simulink library "focLib"  (R2023a)
settings: Solver=VariableStepAuto  StartTime=0.0  StopTime=10.0  RelTol=1e-3
undefined symbols (not defined in the file): availableSpeedModes, ctrl_limits, Down, focp_tune_cur_Ki, focp_tune_cur_Kp, focp_tune_iq_max, focp_tune_iq_min, focp_tune_spd_Ki, focp_tune_spd_Kp, focp_tune_udc_max, GPTRIP1SEL, inverter_DRV8300, PI_params, pmsm_ECI6360, PU_System, target_f2838, Ts, Ts_motor, Ts_simulink, Ts_speed, TZ1, Up
libraries: simulink x31, c2802xlib x12, idelinklib_common x8, mcbcontrolslib x8, c280xlib x7, mcbpositiondecoderlib x7, slpidlib x5, c2837xDlib x2, c2838xlib x1, autolibpmsminterior x1, mcbplantlib x1, autolibpmsmexterior x1
(part 3 of 3)

== system focLib/Torque Controller/FOC/Current_Controllers/PI_Controller_Iq ==
  Iq_in : Inport
  Data Store Read1 : DataStoreRead  Commented=on  DataStoreName=Enable  IndexOptions=Index vector (dialog)  Indices=1  OutputSizes=1
  Discrete PI Controller with anti-windup & reset : slpidlib/PID Controller  Commented=on  Controller=PI  Form=Parallel  TimeDomain=Discrete-time  UseExternalTs=off  SampleTime=-1  IntegratorMethod=Forward Euler  FilterMethod=Forward Euler  ControllerParametersSource=external  P=1  I=1  UseKiTs=on  D=0  N=100  UseFilter=on  TunerSelectOption=Transfer Function Based (PID Tuner App)  InitialConditionSource=external  InitialConditionForIntegrator=0  InitialConditionForFilter=0  DifferentiatorICPrevScaledInput=0  ExternalReset=level  TrackingMode=off  Kt=1  LimitOutput=on  SatLimitsSource=internal  UpperSaturationLimit=1  LowerSaturationLimit=-1  LinearizeAsGain=on  AntiWindupMode=clamping  Kb=1  LimitIntegrator=off  UpperIntegratorSaturationLimit=inf  LowerIntegratorSaturationLimit=-inf  RndMeth=Simplest  POutMin=[]  POutMax=[]  IOutMin=[]  IOutMax=[]  DOutMin=[]  DOutMax=[]  NOutMin=[]  NOutMax=[]  SumOutMin=[]  SumOutMax=[]  SaturationOutDataTypeStr=Inherit: Inherit via back propagation  SaturationOutMin=[]  SaturationOutMax=[]  PParamMin=[]  PParamMax=[]  IParamMin=[]  IParamMax=[]  DParamMin=[]  DParamMax=[]  NParamMin=[]  NParamMax=[]  KbParamMin=[]  KbParamMax=[]  KtParamMin=[]  KtParamMax=[]  KbOutMin=[]  KbOutMax=[]  KtOutMin=[]  KtOutMax=[]  IntegratorOutMin=[]  IntegratorOutMax=[]  FilterOutMin=[]  FilterOutMax=[]  SumI1OutMin=[]  SumI1OutMax=[]  SumI2OutMin=[]  SumI2OutMax=[]  SumI3OutMin=[]  SumI3OutMax=[]  SumI4OutMin=[]  SumI4OutMax=[]  SumDOutMin=[]  SumDOutMax=[]  DifferentiatorOutMin=[]  DifferentiatorOutMax=[]  FilterDiffOutCoefMin=[]  FilterDiffOutCoefMax=[]  ReciprocalOutMin=[]  ReciprocalOutMax=[]  SumDenOutMin=[]  SumDenOutMax=[]  SumNumOutMin=[]  SumNumOutMax=[]  DivideOutMin=[]  DivideOutMax=[]  UdiffTsProdOutMin=[]  UdiffTsProdOutMax=[]  NTsProdOutMin=[]  NTsProdOutMax=[]  UintegralTsProdOutMin=[]  UintegralTsProdOutMax=[]  UngainTsProdOutMin=[]  UngainTsProdOutMax=[]  ClampingZeroOutDataTypeStr=Inherit: Inherit via back propagation  ClampingZeroOutMin=[]  ClampingZeroOutMax=[]  FilterDenConstantOutDataTypeStr=Inherit: Inherit via back propagation  FilterDenConstantOutMin=[]  FilterDenConstantOutMax=[]  PCopyOutDataTypeStr=Inherit: Inherit via back propagation  PCopyOutMin=[]  PCopyOutMax=[]  NCopyOutDataTypeStr=Inherit: Inherit via back propagation  NCopyOutMin=[]  NCopyOutMax=[]  IntegratorContinuousStateAttributes=''  IntegratorStateMustResolveToSignalObject=off  IntegratorRTWStateStorageClass=Auto  FilterContinuousStateAttributes=''  FilterStateMustResolveToSignalObject=off  FilterRTWStateStorageClass=Auto  ParallelPVariant=ExternalParameters  IdealPVariant=Disabled  IVariant=ExternalParameters  DVariant=Disabled  IntegratorVariant=Discrete  SatVariant=Enabled  AWVariant=DiscClampingParallel  PCopyVariant=Disabled  TRVariant=Disabled  FdbkBlocksVariant=Forward  IdealPFdbkVariant=Disabled  SatFdbkVariant=Disabled  DerivativeFilterVariant=Disabled  NVariant=Disabled  NCopyVariant=Disabled_SignalSpec  FilterICVariant=Disabled  IntegratorICVariant=ExternalICs  ExternalResetVariant=ExternalReset  TRSumVariant=Passthrough  SumFdbkVariant=Disabled  SumVariant=Sum_PI  TsampFilterVariant=InternalTs  TsampNgainVariant=Passthrough  TsampIntegralVariant=Disabled_SignalSpec  ExternalSaturationOutDataTypeStr=Inherit: Same as second input
      settings: LibrarySourceBlock=mcbcontrolslib/PI Controller
  Ki : Constant  Commented=on  Value=PI_params.Ki_i*Ts  OutDataTypeStr=single  SampleTime=-1
  Kp : Constant  Commented=on  Value=PI_params.Kp_i  OutDataTypeStr=single  SampleTime=-1
  Kp1 : Constant  Commented=on  Value=0  OutDataTypeStr=single  SampleTime=-1
  Logical Operator : Logic  Commented=on  Operator=NOT  IconShape=distinctive  AllPortsSameDT=off  OutDataTypeStr=boolean
  PID Controller : slpidlib/PID Controller  Controller=PI  Form=Parallel  TimeDomain=Discrete-time  UseExternalTs=off  SampleTime=-1  IntegratorMethod=Forward Euler  FilterMethod=Forward Euler  ControllerParametersSource=internal  P=focp_tune_cur_Kp  I=focp_tune_cur_Ki  UseKiTs=off  D=0  N=100  UseFilter=on  TunerSelectOption=Transfer Function Based (PID Tuner App)  InitialConditionSource=internal  InitialConditionForIntegrator=0  InitialConditionForFilter=0  DifferentiatorICPrevScaledInput=0  ExternalReset=level  TrackingMode=off  Kt=1  LimitOutput=on  SatLimitsSource=internal  UpperSaturationLimit=1  LowerSaturationLimit=-1  LinearizeAsGain=off  AntiWindupMode=clamping  Kb=1  LimitIntegrator=off  UpperIntegratorSaturationLimit=inf  LowerIntegratorSaturationLimit=-inf  POutMin=[]  POutMax=[]  IOutMin=[]  IOutMax=[]  DOutMin=[]  DOutMax=[]  NOutMin=[]  NOutMax=[]  SumOutMin=[]  SumOutMax=[]  SaturationOutMin=[]  SaturationOutMax=[]  PParamDataTypeStr=fixdt(1,32,24)  PParamMin=[]  PParamMax=[]  IParamDataTypeStr=fixdt(1,32,16)  IParamMin=[]  IParamMax=[]  DParamMin=[]  DParamMax=[]  NParamMin=[]  NParamMax=[]  KbParamMin=[]  KbParamMax=[]  KtParamMin=[]  KtParamMax=[]  KbOutMin=[]  KbOutMax=[]  KtOutMin=[]  KtOutMax=[]  IntegratorOutMin=[]  IntegratorOutMax=[]  FilterOutMin=[]  FilterOutMax=[]  SumI1OutMin=[]  SumI1OutMax=[]  SumI2OutMin=[]  SumI2OutMax=[]  SumI3OutMin=[]  SumI3OutMax=[]  SumI4OutMin=[]  SumI4OutMax=[]  SumDOutMin=[]  SumDOutMax=[]  DifferentiatorOutMin=[]  DifferentiatorOutMax=[]  FilterDiffOutCoefMin=[]  FilterDiffOutCoefMax=[]  ReciprocalOutMin=[]  ReciprocalOutMax=[]  SumDenOutMin=[]  SumDenOutMax=[]  SumNumOutMin=[]  SumNumOutMax=[]  DivideOutMin=[]  DivideOutMax=[]  UdiffTsProdOutMin=[]  UdiffTsProdOutMax=[]  NTsProdOutMin=[]  NTsProdOutMax=[]  UintegralTsProdOutMin=[]  UintegralTsProdOutMax=[]  UngainTsProdOutMin=[]  UngainTsProdOutMax=[]  ClampingZeroOutDataTypeStr=Inherit: Inherit via back propagation  ClampingZeroOutMin=[]  ClampingZeroOutMax=[]  FilterDenConstantOutDataTypeStr=Inherit: Inherit via back propagation  FilterDenConstantOutMin=[]  FilterDenConstantOutMax=[]  PCopyOutDataTypeStr=Inherit: Inherit via back propagation  PCopyOutMin=[]  PCopyOutMax=[]  NCopyOutDataTypeStr=Inherit: Inherit via back propagation  NCopyOutMin=[]  NCopyOutMax=[]  IntegratorContinuousStateAttributes=''  IntegratorStateMustResolveToSignalObject=off  IntegratorRTWStateStorageClass=Auto  FilterContinuousStateAttributes=''  FilterStateMustResolveToSignalObject=off  FilterRTWStateStorageClass=Auto  ParallelPVariant=InternalParameters  IdealPVariant=Disabled  IVariant=InternalParameters  DVariant=Disabled  IntegratorVariant=Discrete  SatVariant=Enabled  AWVariant=DiscClampingParallel  PCopyVariant=Disabled  TRVariant=Disabled  FdbkBlocksVariant=Forward  IdealPFdbkVariant=Disabled  SatFdbkVariant=Disabled  DerivativeFilterVariant=Disabled  NVariant=Disabled  NCopyVariant=Disabled_SignalSpec  FilterICVariant=Disabled  IntegratorICVariant=InternalICs  ExternalResetVariant=ExternalReset  TRSumVariant=Passthrough  SumFdbkVariant=Disabled  SumVariant=Sum_PI  TsampFilterVariant=InternalTs  TsampNgainVariant=Passthrough  TsampIntegralVariant=Disabled_SignalSpec  ExternalSaturationOutDataTypeStr=Inherit: Same as second input
  Reset_I_Cur_And : Logic  AllPortsSameDT=off  OutDataTypeStr=boolean
  Reset_I_Cur_Enable : Constant  Value=ctrl_limits.reset_I_cur_freemode  OutDataTypeStr=boolean
  V_ref : Outport  VectorParamsAs1DForOutWhenUnconnected=off
  wires:
  Iq_in/1 -> PID Controller/1
  PID Controller/1 -> V_ref/1
  Kp1/1 -> Discrete PI Controller with anti-windup & reset/5
  Logical Operator/1 -> Discrete PI Controller with anti-windup & reset/4
  Ki/1 -> Discrete PI Controller with anti-windup & reset/3
  Kp/1 -> Discrete PI Controller with anti-windup & reset/2
  Data Store Read1/1 -> Logical Operator/1
  [FreemodeSig_I] -> Reset_I_Cur_And/1
  Reset_I_Cur_Enable/1 -> Reset_I_Cur_And/2
  Reset_I_Cur_And/1 -> PID Controller/2

== system focLib/Torque Controller/Input Scaling/CodeGeneration/Calculate Position from Hall ==
  Atomic Hall Reading : Subsystem
  Data Store Write : DataStoreWrite  DataStoreName=HallStateChangeFlag  IndexOptions=Index vector (dialog)  Indices=1  OutputSizes=1
  Glitch Filter : simulink/Logic and Bit Operations/Compare To Constant  relop=>=  const=target_f2838.CPU_frequency * 600 / (pmsm_ECI6360.N_base * 10 * 2 * pmsm_ECI6360.p)  OutDataTypeStr=boolean
  Hall Speed and Position : mcbpositiondecoderlib/Hall Speed and Position  blkExecutionType=Speed and position  CounterSize=32 bits  ClkFreq=target_f2838.CPU_frequency  BlkSampleTime=Ts  PolePairs=pmsm_ECI6360.p  MinSpeed=20  HallInterruptConfig=Every 180 Degrees  SpeedUnit=Per unit  PerUnitSpeed=PU_System.N_base  SpeedDataType=fixdt(1,32,17)  hallSequence=ABC  Sequence=[5,4,6,2,3,1]  EnableSecondOrder=1st Order  PositionUnit=Per unit  PositionDataType=fixdt(1,32,17)
      settings: LibrarySourceBlock=mcblib/Sensor Decoders/Hall Speed and Position
  Mechanical to Electrical Position : mcbpositiondecoderlib/Mechanical to Electrical Position  NrPP=1  selectedRange=Per unit  MechOfstInputType=Specify via dialog  mechOffsetIn=0.38  maxAngleIn=1  InputDataType=fixdt(1,32,17)  VariantSelect=floating-point
      settings: LibrarySourceBlock=mcblib/Sensor Decoders/Mechanical to Electrical Position
  Subsystem : Subsystem
  Pos_PU : Outport
  Speed_PU : Outport  Port=2
  wires:
  Hall Speed and Position/2 -> Speed_PU/1
  Subsystem/1(Output) -> Hall Speed and Position/3
  Atomic Hall Reading/3(SpeedCount) -> Glitch Filter/1, Subsystem/1(Input)
  Glitch Filter/1 -> Subsystem/Enable
  Mechanical to Electrical Position/1 -> Pos_PU/1
  Hall Speed and Position/1 -> Mechanical to Electrical Position/1
  Atomic Hall Reading/1(HallState) -> Hall Speed and Position/1
  Atomic Hall Reading/4(Direction) -> Hall Speed and Position/4
  Atomic Hall Reading/2(Count) -> Hall Speed and Position/2
  Atomic Hall Reading/5(SpeedValidity) -> Hall Speed and Position/5
  Hall Speed and Position/3 -> Data Store Write/1
  Atomic Hall Reading/6(HallChange) -> Hall Speed and Position/6

== system focLib/Torque Controller/Input Scaling/CodeGeneration/Convert ADC value to PU ==
  note: Shift Gain mit 2hoch9 und fixdt(1,32,20) einmal versuchen
  Iab_ADC : Inport
  Add : Sum  Inputs=+-
  Data Store Read : DataStoreRead  DataStoreName=IaOffset  IndexOptions=Index vector (dialog)  Indices=1  OutputSizes=1
  Data Store Read1 : DataStoreRead  DataStoreName=IbOffset  IndexOptions=Index vector (dialog)  Indices=1  OutputSizes=1
  Data Type Conversion : DataTypeConversion  OutDataTypeStr=int32  ConvertRealWorld=Stored Integer (SI)  SaturateOnIntegerOverflow=off  RndMeth=Floor
  Data Type Conversion1 : DataTypeConversion  OutDataTypeStr=fixdt(1,32,17)  ConvertRealWorld=Stored Integer (SI)  SaturateOnIntegerOverflow=off  RndMeth=Floor
  Display{,1..3} (4 alike) : Display
  Mux : Mux  Inputs=2
  Shift Arithmetic : ArithShift  BitShiftNumber=-6
  Iab_PU : Outport
  wires:
  Data Store Read1/1 -> Mux/2
  Data Store Read/1 -> Mux/1
  Data Type Conversion1/1 -> Display/1, Iab_PU/1
  Shift Arithmetic/1 -> Data Type Conversion1/1, Display1/1
  Add/1 -> Shift Arithmetic/1, Display2/1
  Mux/1 -> Add/2
  Data Type Conversion/1 -> Add/1, Display3/1
  Iab_ADC/1 -> Data Type Conversion/1

== system focLib/Torque Controller/Input Scaling/Simulation/Convert Iab to PU ==
  Iab_ADC_Sim : Inport
  Add : Sum  Inputs=+-
  Constant : Constant  Value=[inverter_DRV8300.CtSensAOffset inverter_DRV8300.CtSensBOffset]  SampleTime=-1
  Current Sense Gain : Gain  Commented=on  Gain=PU_System.I_base/1.65  RndMeth=Simplest  OutDataTypeStr=Inherit: Same as input
  Data Type Conversion : DataTypeConversion  OutDataTypeStr=int32  ConvertRealWorld=Stored Integer (SI)  SaturateOnIntegerOverflow=off  RndMeth=Floor
  Data Type Conversion1 : DataTypeConversion  OutDataTypeStr=fixdt(1,32,17)  ConvertRealWorld=Stored Integer (SI)  RndMeth=Simplest  SaturateOnIntegerOverflow=off
  Get_ADC_Volt : Gain  Commented=on  Gain=1.65/(4096/2)  OutDataTypeStr=double  RndMeth=Simplest
  PU_Conversion : Gain  Commented=on  Gain=1/PU_System.I_base  RndMeth=Simplest  OutDataTypeStr=Inherit: Same as input
  Shift Arithmetic : ArithShift  BitShiftNumber=-6
  Iab_PU : Outport
  wires:
  Get_ADC_Volt/1 -> Current Sense Gain/1
  Current Sense Gain/1 -> PU_Conversion/1
  Add/1 -> Shift Arithmetic/1
  Shift Arithmetic/1 -> Data Type Conversion1/1
  Data Type Conversion1/1 -> Iab_PU/1
  Constant/1 -> Add/2
  Data Type Conversion/1 -> Add/1
  Iab_ADC_Sim/1 -> Data Type Conversion/1

== system focLib/Torque Controller/Input Scaling/Simulation/Convert Pos to PU ==
  Pos_Sim : Inport
  IIR Filter : mcbcontrolslib/IIR Filter  VariantControl=Low Pass Filter  VariantSelect=Low-pass  Filter_constant=0.2  advancedSettings=off  Ts=50e-6  cutOff_freq=795.7747
      settings: LibrarySourceBlock=mcbhdllib/Signal Management/IIR Filter
  Mechanical to Electrical Position : mcbpositiondecoderlib/Mechanical to Electrical Position  NrPP=pmsm_ECI6360.p  selectedRange=Per unit  MechOfstInputType=Specify via dialog  mechOffsetIn=0.38  maxAngleIn=1  InputDataType=fixdt(1,32,17)  VariantSelect=floating-point
      settings: LibrarySourceBlock=mcblib/Sensor Decoders/Mechanical to Electrical Position
  Speed Measurement : mcbpositiondecoderlib/Speed Measurement  PositionUnit=Per unit  PositionScalingDatatype=uint32  SpeedCalculationMode=Time interval for speed calculation  SampleTimeAsync=Ts  MaximumApplicationSpeed=1000  SpeedResolution=5e-6  DelayLength=10  MaximumMeasurableSpeed=59999  MeasurableSpeedResolution=2.794e-05  SpeedUnit=Per unit based on dialog  PerUnitSpeed=PU_System.N_base  SpeedDataType=fixdt(1,32,17)
      settings: LibrarySourceBlock=mcblib/Sensor Decoders/Speed Measurement
  Theta : Outport
  Speed_PU : Outport  Port=2
  wires:
  IIR Filter/1 -> Speed_PU/1
  Mechanical to Electrical Position/1 -> Theta/1
  Speed Measurement/1 -> IIR Filter/1
  Pos_Sim/1 -> Speed Measurement/1, Mechanical to Electrical Position/1

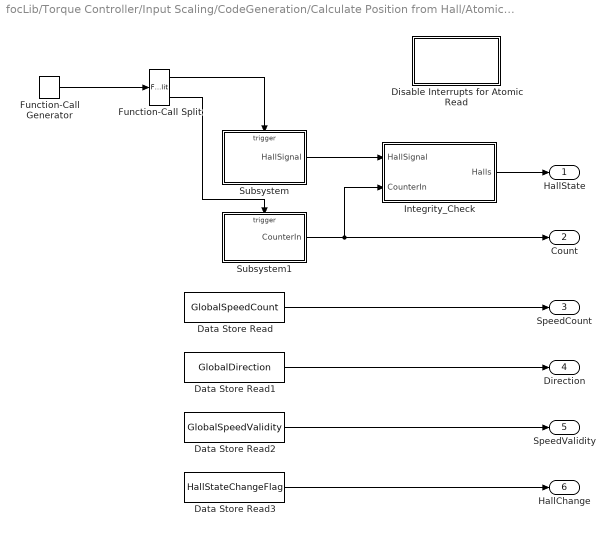
== system focLib/Torque Controller/Input Scaling/CodeGeneration/Calculate Position from Hall/Atomic Hall Reading ==
  Data Store Read : DataStoreRead  DataStoreName=GlobalSpeedCount  IndexOptions=Index vector (dialog)  Indices=1  OutputSizes=1
  Data Store Read1 : DataStoreRead  DataStoreName=GlobalDirection  IndexOptions=Index vector (dialog)  Indices=1  OutputSizes=1
  Data Store Read2 : DataStoreRead  DataStoreName=GlobalSpeedValidity  IndexOptions=Index vector (dialog)  Indices=1  OutputSizes=1
  Data Store Read3 : DataStoreRead  DataStoreName=HallStateChangeFlag  IndexOptions=Index vector (dialog)  Indices=1  OutputSizes=1
  Disable Interrupts for Atomic Read : Subsystem  mask(System Outputs){ShowInLibBrowser=0}
      mask prompts: ShowInLibBrowser "Simulink:masks:CustCodeMaskParam1_MP"
      settings: CopyFcn=cccopyfcn(gcb)  OpenFcn=ccopenfcn('System Outputs Function')
      mask Help: eval('feval(''rtwprivate'',''rtwhelpview'',''rtw_sys_outputs_block'')');
      mask Display: disp('System\nOutputs');
  Function-Call Generator : simulink/Ports & Subsystems/Function-Call Generator  sample_time=-1  numberOfIterations=1  DisallowWideOutput=off
  Function-Call Split : FunctionCallSplit  IconShape=distinctive  NumOutputPorts=2  OutputPortLayout=default
  Integrity_Check : Subsystem
  Subsystem : Subsystem
  Subsystem1 : Subsystem
  HallState : Outport
  Count : Outport  Port=2
  SpeedCount : Outport  Port=3
  Direction : Outport  Port=4
  SpeedValidity : Outport  Port=5
  HallChange : Outport  Port=6
  wires:
  Subsystem1/1(CounterIn) -> Integrity_Check/2(CounterIn), Count/1
  Function-Call Split/1 -> Subsystem/Trigger
  Function-Call Split/2 -> Subsystem1/Trigger
  Integrity_Check/1(Halls) -> HallState/1
  Subsystem/1(HallSignal) -> Integrity_Check/1(HallSignal)
  Data Store Read/1 -> SpeedCount/1
  Data Store Read1/1 -> Direction/1
  Data Store Read3/1 -> HallChange/1
  Data Store Read2/1 -> SpeedValidity/1
  Function-Call Generator/1 -> Function-Call Split/1

== system focLib/Torque Controller/Input Scaling/CodeGeneration/Calculate Position from Hall/Subsystem ==
  Input : Inport
  Enable : EnablePort
  Output : Outport
  wires:
  Input/1 -> Output/1

== system focLib/Torque Controller/Input Scaling/CodeGeneration/Calculate Position from Hall/Atomic Hall Reading/Disable Interrupts for Atomic Read ==

== system focLib/Torque Controller/Input Scaling/CodeGeneration/Calculate Position from Hall/Atomic Hall Reading/Integrity_Check ==
  HallSignal : Inport
  CounterIn : Inport  Port=2
  Compare To Constant : simulink/Logic and Bit Operations/Compare To Constant  relop=<=  const=2500  OutDataTypeStr=boolean
  Display1 : Display
  If : If  IfExpression=u1 == 0
  Merge : Merge
  NOT : Logic  AllPortsSameDT=off  OutDataTypeStr=boolean
  No_Integrity_issue : Subsystem  TreatAsAtomicUnit=on
  Refresh_Halls : Subsystem  TreatAsAtomicUnit=on
  Relational Operator : RelationalOperator  Operator===  OutDataTypeStr=boolean  RndMeth=Simplest  InputSameDT=off
  Unit Delay : UnitDelay  SampleTime=-1  HasFrameUpgradeWarning=on
  Halls : Outport
  wires:
  Unit Delay/1 -> Relational Operator/2
  NOT/1 -> If/1
  Relational Operator/1 -> NOT/1
  Compare To Constant/1 -> NOT/2
  CounterIn/1 -> Compare To Constant/1
  If/1 -> No_Integrity_issue/Action
  No_Integrity_issue/1(Out1) -> Merge/1
  Merge/1 -> Halls/1
  If/2 -> Refresh_Halls/Action
  HallSignal/1 -> Unit Delay/1, No_Integrity_issue/1(Counter), Relational Operator/1, Display1/1
  Refresh_Halls/1(Out1) -> Merge/2

== system focLib/Torque Controller/Input Scaling/CodeGeneration/Calculate Position from Hall/Atomic Hall Reading/Subsystem ==
  function call : TriggerPort  TriggerType=function-call  VariantControl=(inherit)  PortDimensions=1
  Bitwise OR : simulink/Logic and Bit Operations/Bitwise Operator  logicop=OR  UseBitMask=off  NumInputPorts=3  BitMask=bin2dec('11011001')  BitMaskRealWorld=Stored Integer
      settings: LibrarySourceBlock=|
      | simulink/Quick Insert/Logic and Bit
      | Operations/Bitwise OR
  Data Type Conversion : DataTypeConversion  OutDataTypeStr=uint32  ConvertRealWorld=Stored Integer (SI)  SaturateOnIntegerOverflow=off  RndMeth=Floor
  GPIO 24 Hall_A : simulink/Logic and Bit Operations/Bitwise Operator  logicop=AND  UseBitMask=on  BitMask=hex2dec('1000000')  BitMaskRealWorld=Stored Integer
      settings: LibrarySourceBlock=|
      | simulink/Quick Insert/Logic and Bit
      | Operations/Bitwise AND
  GPIO 25 Hall_B : simulink/Logic and Bit Operations/Bitwise Operator  logicop=AND  UseBitMask=on  BitMask=hex2dec('2000000')  BitMaskRealWorld=Stored Integer
      settings: LibrarySourceBlock=|
      | simulink/Quick Insert/Logic and Bit
      | Operations/Bitwise AND
  GPIO 26 Hall_C : simulink/Logic and Bit Operations/Bitwise Operator  logicop=AND  UseBitMask=on  BitMask=hex2dec('4000000')  BitMaskRealWorld=Stored Integer
      settings: LibrarySourceBlock=|
      | simulink/Quick Insert/Logic and Bit
      | Operations/Bitwise AND
  Memory Copy : idelinklib_common/Memory Copy  copyFrom=Specified source code symbol  copyFromAddressSource=Specify via dialog  copyFromAddress=hex2dec('00001000')  copyFromSrcCode=&GpioDataRegs.GPADAT.all  dataTypeFrom=uint32  dataDimensionFrom=1  useOffsetFrom=off  offsetFromSrc=Specify via dialog  offsetFrom=0  strideFrom=1  copyTo=Output port  copyToAddressSource=Specify via dialog  copyToAddress=hex2dec('00002000')  copyToSrcCode=myVariableDst  dataTypeTo=uint32  useOffsetTo=off  offsetToSrc=Specify via dialog  offsetTo=0  strideTo=1  sampleTime=-1  useInitValue=off  initValueSrc=Specify constant value  initValue=1  initValueSrcCode=myInitValueVariable  useAsMask=off  maskOperator=bitwise AND  useTermValue=off  termValue=1  isRealtimeEnabled=off  emitCCBeforeWrite=off  CCBeforeWrite=/* Custom Code Before Write*/  emitCCAfterWrite=off  CCAfterWrite=/* Custom Code After Write*/
  Shift Arithmetic : ArithShift  BitShiftNumber=26
  Shift Arithmetic1 : ArithShift  BitShiftNumber=24
  Shift Arithmetic2 : ArithShift  BitShiftNumber=22
  HallSignal : Outport
  wires:
  GPIO 26 Hall_C/1 -> Shift Arithmetic/1
  GPIO 25 Hall_B/1 -> Shift Arithmetic1/1
  GPIO 24 Hall_A/1 -> Shift Arithmetic2/1
  Bitwise OR/1 -> Data Type Conversion/1
  Shift Arithmetic/1 -> Bitwise OR/1
  Memory Copy/1 -> GPIO 25 Hall_B/1, GPIO 26 Hall_C/1, GPIO 24 Hall_A/1
  Shift Arithmetic1/1 -> Bitwise OR/2
  Shift Arithmetic2/1 -> Bitwise OR/3
  Data Type Conversion/1 -> HallSignal/1

== system focLib/Torque Controller/Input Scaling/CodeGeneration/Calculate Position from Hall/Atomic Hall Reading/Subsystem1 ==
  function-call : TriggerPort  TriggerType=function-call  VariantControl=(inherit)  PortDimensions=1
  Memory Copy : idelinklib_common/Memory Copy  copyFrom=Specified source code symbol  copyFromAddressSource=Specify via dialog  copyFromAddress=hex2dec('00001000')  copyFromSrcCode=&ECap1Regs.TSCTR  dataTypeFrom=uint32  dataDimensionFrom=1  useOffsetFrom=off  offsetFromSrc=Specify via dialog  offsetFrom=0  strideFrom=1  copyTo=Output port  copyToAddressSource=Specify via dialog  copyToAddress=hex2dec('00002000')  copyToSrcCode=myVariableDst  dataTypeTo=uint32  useOffsetTo=off  offsetToSrc=Specify via dialog  offsetTo=0  strideTo=1  sampleTime=-1  useInitValue=off  initValueSrc=Specify constant value  initValue=1  initValueSrcCode=myInitValueVariable  useAsMask=off  maskOperator=bitwise AND  useTermValue=off  termValue=1  isRealtimeEnabled=off  emitCCBeforeWrite=off  CCBeforeWrite=/* Custom Code Before Write*/  emitCCAfterWrite=off  CCAfterWrite=/* Custom Code After Write*/
  Memory Copy1 : idelinklib_common/Memory Copy  copyFrom=Specified source code symbol  copyFromAddressSource=Specify via dialog  copyFromAddress=hex2dec('00001000')  copyFromSrcCode=&ECap2Regs.TSCTR  dataTypeFrom=uint32  dataDimensionFrom=1  useOffsetFrom=off  offsetFromSrc=Specify via dialog  offsetFrom=0  strideFrom=1  copyTo=Output port  copyToAddressSource=Specify via dialog  copyToAddress=hex2dec('00002000')  copyToSrcCode=myVariableDst  dataTypeTo=uint32  useOffsetTo=off  offsetToSrc=Specify via dialog  offsetTo=0  strideTo=1  sampleTime=-1  useInitValue=off  initValueSrc=Specify constant value  initValue=1  initValueSrcCode=myInitValueVariable  useAsMask=off  maskOperator=bitwise AND  useTermValue=off  termValue=1  isRealtimeEnabled=off  emitCCBeforeWrite=off  CCBeforeWrite=/* Custom Code Before Write*/  emitCCAfterWrite=off  CCAfterWrite=/* Custom Code After Write*/
  Memory Copy2 : idelinklib_common/Memory Copy  copyFrom=Specified source code symbol  copyFromAddressSource=Specify via dialog  copyFromAddress=hex2dec('00001000')  copyFromSrcCode=&ECap3Regs.TSCTR  dataTypeFrom=uint32  dataDimensionFrom=1  useOffsetFrom=off  offsetFromSrc=Specify via dialog  offsetFrom=0  strideFrom=1  copyTo=Output port  copyToAddressSource=Specify via dialog  copyToAddress=hex2dec('00002000')  copyToSrcCode=myVariableDst  dataTypeTo=uint32  useOffsetTo=off  offsetToSrc=Specify via dialog  offsetTo=0  strideTo=1  sampleTime=-1  useInitValue=off  initValueSrc=Specify constant value  initValue=1  initValueSrcCode=myInitValueVariable  useAsMask=off  maskOperator=bitwise AND  useTermValue=off  termValue=1  isRealtimeEnabled=off  emitCCBeforeWrite=off  CCBeforeWrite=/* Custom Code Before Write*/  emitCCAfterWrite=off  CCAfterWrite=/* Custom Code After Write*/
  Min : MinMax  Inputs=3
  CounterIn : Outport
  wires:
  Memory Copy2/1 -> Min/3
  Memory Copy/1 -> Min/1
  Min/1 -> CounterIn/1
  Memory Copy1/1 -> Min/2

== system focLib/Torque Controller/Input Scaling/CodeGeneration/Calculate Position from Hall/Atomic Hall Reading/Integrity_Check/No_Integrity_issue ==
  Counter : Inport
  Action Port : ActionPort
  Out1 : Outport
  wires:
  Counter/1 -> Out1/1

== system focLib/Torque Controller/Input Scaling/CodeGeneration/Calculate Position from Hall/Atomic Hall Reading/Integrity_Check/Refresh_Halls ==
  Action Port : ActionPort
  Bitwise OR : simulink/Logic and Bit Operations/Bitwise Operator  logicop=OR  UseBitMask=off  NumInputPorts=3  BitMask=bin2dec('11011001')  BitMaskRealWorld=Stored Integer
      settings: LibrarySourceBlock=|
      | simulink/Quick Insert/Logic and Bit
      | Operations/Bitwise OR
  Data Type Conversion : DataTypeConversion  OutDataTypeStr=uint32  ConvertRealWorld=Stored Integer (SI)  SaturateOnIntegerOverflow=off  RndMeth=Floor
  GPIO 24 Hall_A : simulink/Logic and Bit Operations/Bitwise Operator  logicop=AND  UseBitMask=on  BitMask=hex2dec('1000000')  BitMaskRealWorld=Stored Integer
      settings: LibrarySourceBlock=|
      | simulink/Quick Insert/Logic and Bit
      | Operations/Bitwise AND
  GPIO 25 Hall_B : simulink/Logic and Bit Operations/Bitwise Operator  logicop=AND  UseBitMask=on  BitMask=hex2dec('2000000')  BitMaskRealWorld=Stored Integer
      settings: LibrarySourceBlock=|
      | simulink/Quick Insert/Logic and Bit
      | Operations/Bitwise AND
  GPIO 26 Hall_C : simulink/Logic and Bit Operations/Bitwise Operator  logicop=AND  UseBitMask=on  BitMask=hex2dec('4000000')  BitMaskRealWorld=Stored Integer
      settings: LibrarySourceBlock=|
      | simulink/Quick Insert/Logic and Bit
      | Operations/Bitwise AND
  Memory Copy : idelinklib_common/Memory Copy  copyFrom=Specified source code symbol  copyFromAddressSource=Specify via dialog  copyFromAddress=hex2dec('00001000')  copyFromSrcCode=&GpioDataRegs.GPADAT.all  dataTypeFrom=uint32  dataDimensionFrom=1  useOffsetFrom=off  offsetFromSrc=Specify via dialog  offsetFrom=0  strideFrom=1  copyTo=Output port  copyToAddressSource=Specify via dialog  copyToAddress=hex2dec('00002000')  copyToSrcCode=myVariableDst  dataTypeTo=uint32  useOffsetTo=off  offsetToSrc=Specify via dialog  offsetTo=0  strideTo=1  sampleTime=-1  useInitValue=off  initValueSrc=Specify constant value  initValue=1  initValueSrcCode=myInitValueVariable  useAsMask=off  maskOperator=bitwise AND  useTermValue=off  termValue=1  isRealtimeEnabled=off  emitCCBeforeWrite=off  CCBeforeWrite=/* Custom Code Before Write*/  emitCCAfterWrite=off  CCAfterWrite=/* Custom Code After Write*/
  Shift Arithmetic : ArithShift  BitShiftNumber=26
  Shift Arithmetic1 : ArithShift  BitShiftNumber=24
  Shift Arithmetic2 : ArithShift  BitShiftNumber=22
  Out1 : Outport
  wires:
  GPIO 26 Hall_C/1 -> Shift Arithmetic/1
  GPIO 24 Hall_A/1 -> Shift Arithmetic2/1
  Bitwise OR/1 -> Data Type Conversion/1
  Shift Arithmetic/1 -> Bitwise OR/1
  Memory Copy/1 -> GPIO 25 Hall_B/1, GPIO 24 Hall_A/1, GPIO 26 Hall_C/1
  GPIO 25 Hall_B/1 -> Shift Arithmetic1/1
  Shift Arithmetic1/1 -> Bitwise OR/2
  Shift Arithmetic2/1 -> Bitwise OR/3
  Data Type Conversion/1 -> Out1/1

== matlab function focLib/Torque Controller/FOC/FOCP ISR ==
  data: iab input single size=2; pos input single; idq input single size=2; vdq input single size=2; ic_raw input uint16
function focp_isr(iab, pos, idq, vdq, ic_raw)
% FOCP-Telemetrie und Schutz im Stromregler-Interrupt, nur im erzeugten Code (firmware/focp_c28x.c).
if coder.target('Rtw')
    coder.cinclude('focp_c28x.h');
    coder.ceval('focp_c28x_isr', coder.rref(iab), pos, coder.rref(idq), coder.rref(vdq), ic_raw);
end
end
